simulink model "lab3_pendulum"  (R2023a)
settings: Solver=ode45  StartTime=0.0  StopTime=10  MaxStep=0.01  RelTol=1e-8
InitFcn:
  | d = struct('g',9.81,'l',1,'m',1,'K1',0,'K2',0,'Fm',0,'Om',2,'phi0',0.5);f = fieldnames(d);for k = 1:numel(f),   if ~evalin('base',['exist(''' f{k} ''',''var'')']),     assignin('base',f{k},d.(f{k}));   end; end
values from neighbouring files (symbols this model uses):
  phi0 = 0.5    [lab3_all_figures_from_simulink.m]
undefined symbols (not defined in the file or in its folder): Fm, g, K1, K2, l, m, Om
settings Model: Creator=maybn  LastModifiedBy=maybn

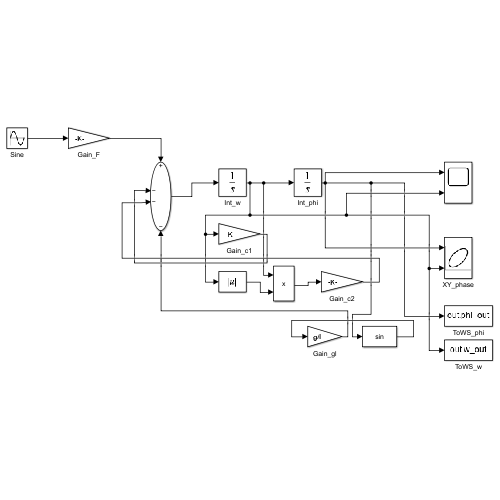
[thumbnail: Simulink's stored preview of the top-level diagram]
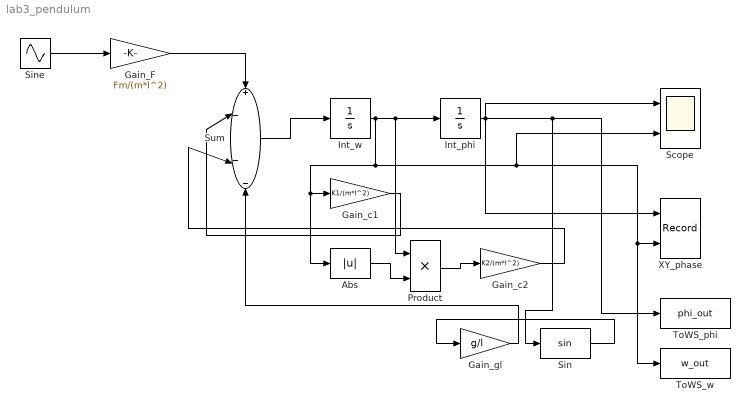
== system lab3_pendulum ==
  Abs : Abs  SaturateOnIntegerOverflow=off
  Gain_F : Gain  Gain=Fm/(m*l^2)
  Gain_c1 : Gain  Gain=K1/(m*l^2)
  Gain_c2 : Gain  Gain=K2/(m*l^2)
  Gain_gl : Gain  Gain=g/l
  Int_phi : Integrator  InitialCondition=phi0
  Int_w : Integrator
  Product : Product
  Scope : Scope  NumInputPorts=2
  Sin : Trigonometry
  Sine : Sin  Frequency=Om  SampleTime=0
  Sum : Sum  Inputs=+---
  ToWS_phi : ToWorkspace  VariableName=phi_out  SampleTime=-1
  ToWS_w : ToWorkspace  VariableName=w_out  SampleTime=-1
  XY_phase : Record  FileSettingsInternal="{\"entries\":[{\"content\":{\"excelSettings\":{\"content\":{},\"type\":\"Streamout.ExcelSettings\"}},\"type\":\"Streamout.FileSettingStorage\",\"uuid\":\"e3aa02d6-b7a0-4234-8bfd-15472c44c14a\"}],\"packageUris\":[\"http://schema.mathworks.com/mf0/streamout_blocks/R2020a\"],\"version\":\"1.0\"}"  Layout=[1 1]  SignalsInternal="{\"entries\":[{\"content\":{\"signals\":[{\"content\":{\"blockPath\":[\"lab3_pendulum/XY_phase\"],\"dimensions\":[1],\"domain\":\"lab3_pendulum/XY_phase\",\"lineColor\":\"#a2142f\",\"plots\":[1],\"port\":1,\"signalID\":142,\"signalName\":\"XY Graph:1\"},\"type\":\"RecordBlkView.Signal\",\"uuid\":\"e207c869-bb8d-4f46-8b05-bd5810cf13b4\"},{\"content\":{\"blockPath\":[\"lab3_pendulum/XY_phase\"],\"dimensions\":[1],\"domain\":\"lab3_pendulum/XY_phase\",\"lineColor\":\"#139fff\",\"plots\":[1],\"port\":2,\"signalID\":145,\"signalName\":\"XY Graph:2\"},\"type\":\"RecordBlkView.Signal\",\"uuid\":\"beb84717-4208-4950-bd00-18678478704f\"}]},\"type\":\"RecordBlkView.InputSignals\",\"uuid\":\"3f31aae7-cfa6-4e7c-bb83-8175eedccb38\"}],\"packageUris\":[\"http://schema.mathworks.com/mf0/streamout_blocks/R2020a\"],\"version\":\"1.0\"}"  VisualizationBindings="{\"xyplotplugin\":{\"info\":[{\"series\":[{\"bindingParametersList\":[{\"parameter\":\"X-Axis\",\"signalID\":142,\"signalName\":\"XY Graph:1\"},{\"parameter\":\"Y-Axis\",\"signalID\":145,\"signalName\":\"XY Graph:2\"}],\"seriesID\":2143}],\"subplotID\":1}]}}"  CompatibilityTag=XY
  wires:
  Sine/1 -> Gain_F/1
  Gain_F/1 -> Sum/1
  Sum/1 -> Int_w/1
  Int_w/1 -> ToWS_w/1, XY_phase/2, Scope/2, Gain_c1/1, Abs/1, Int_phi/1, Product/1
  Gain_c1/1 -> Sum/2
  Abs/1 -> Product/2
  Product/1 -> Gain_c2/1
  Gain_c2/1 -> Sum/3
  Int_phi/1 -> Sin/1, ToWS_phi/1, Scope/1, XY_phase/1
  Sin/1 -> Gain_gl/1
  Gain_gl/1 -> Sum/4
